simulink model "BEV_Components_OctNov24"  (R2024b)
settings: Solver=ode23tb  StartTime=0.0  StopTime=50  RelTol=1e-3
InitFcn:
  | P=150;
  | i_g=20;
  | Batt_C=90;
  | 
  | m=1200;
  | c=.28;
  | frr=0.014;
  | g=9.81;
  | Cmax=Batt_C*1e3/340;
  | et=0.9;
  | rw=.37;
libraries: simulink x1
settings Model: Creator=Kamyar  LastModifiedBy=samar
settings SolverCC: AlgebraicLoopSolver=TrustRegion
settings DebuggingCC: UnconnectedInputMsg=warning  UnconnectedOutputMsg=warning  UnconnectedLineMsg=warning
settings ModelReferenceCC: EnableRefExpFcnMdlSchedulingChecks=on
settings RTWCC: GPUComputeCapability=3.5  DLArmComputeVersion=19.05

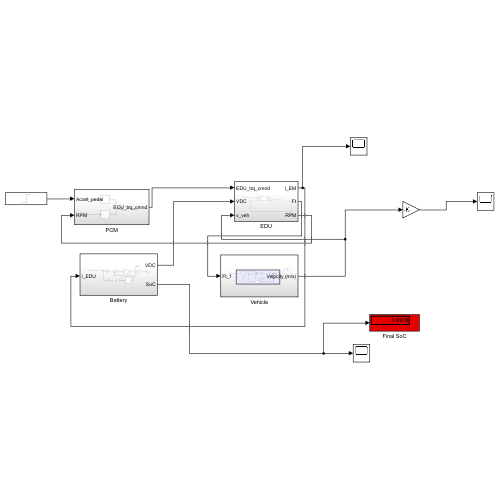
[thumbnail: Simulink's stored preview of the top-level diagram]
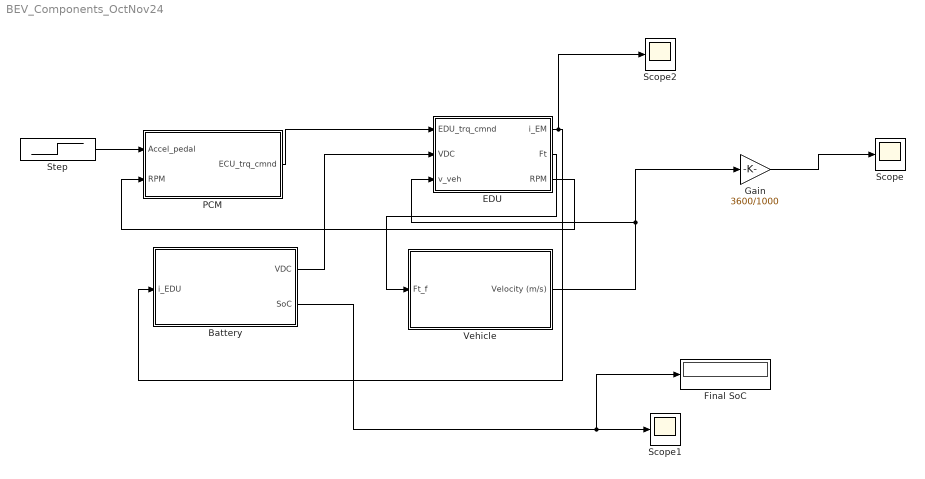
== system BEV_Components_OctNov24 ==
  Battery : Subsystem
  EDU : Subsystem
  Final SoC : Display
  Gain : Gain  Gain=3600/1000
  PCM : Subsystem
  Scope : Scope
  Scope1 : Scope
  Scope2 : Scope
  Step : Step  After=.6  SampleTime=0
  Vehicle : Subsystem
  wires:
  PCM/1(ECU_trq_cmnd) -> EDU/1(EDU_trq_cmnd)
  EDU/3(RPM) -> PCM/2(RPM)
  EDU/1(i_EM) -> Scope2/1, Battery/1(i_EDU)
  EDU/2(Ft) -> Vehicle/1(Ft_f)
  Battery/1(VDC) -> EDU/2(VDC)
  Vehicle/1(Velocity (m/s)) -> Gain/1, EDU/3(v_veh)
  Step/1 -> PCM/1(Accel_pedal)
  Battery/2(SoC) -> Final SoC/1, Scope1/1
  Gain/1 -> Scope/1

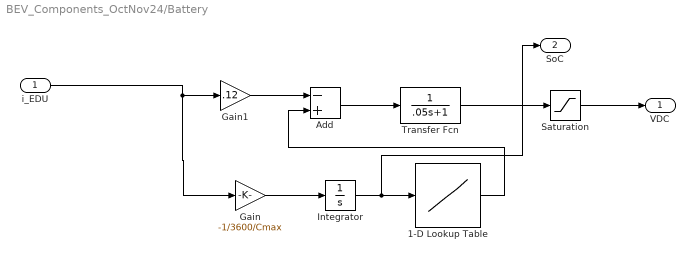
== system BEV_Components_OctNov24/Battery ==
  i_EDU : Inport
  1-D Lookup Table : Lookup_n-D  NumberOfTableDimensions=1  BreakpointsForDimension1=|  Table=|  InternalRulePriority=Speed  RndMeth=Simplest
      BreakpointsForDimension1=|
      | [0
      | 0.028708134
      | 0.04784689
      | 0.105263158
      | 0.207336523
      | 0.398724083
      | 0.535885167
      | 0.596491228
      | 0.68261563
      | 0.797448166
      | 1
      | ]
      Table=|
      | [279.7468354
      | 298.9873418
      | 313.164557
      | 323.0379747
      | 330.6329114
      | 339.7468354
      | 344.556962
      | 347.8481013
      | 356.4556962
      | 367.0886076
      | 391.1392405
      | ]
  Add : Sum  Inputs=-+
  Gain : Gain  Gain=-1/3600/Cmax
  Gain1 : Gain  Gain=.12
  Integrator : Integrator  InitialCondition=1
  Saturation : Saturate  UpperLimit=inf  LowerLimit=200
  Transfer Fcn : TransferFcn  Denominator=[.05 1]
  VDC : Outport
  SoC : Outport  Port=2
  wires:
  i_EDU/1 -> Gain/1, Gain1/1
  Gain/1 -> Integrator/1
  Integrator/1 -> SoC/1, 1-D Lookup Table/1
  1-D Lookup Table/1 -> Add/2
  Gain1/1 -> Add/1
  Add/1 -> Transfer Fcn/1
  Transfer Fcn/1 -> Saturation/1
  Saturation/1 -> VDC/1

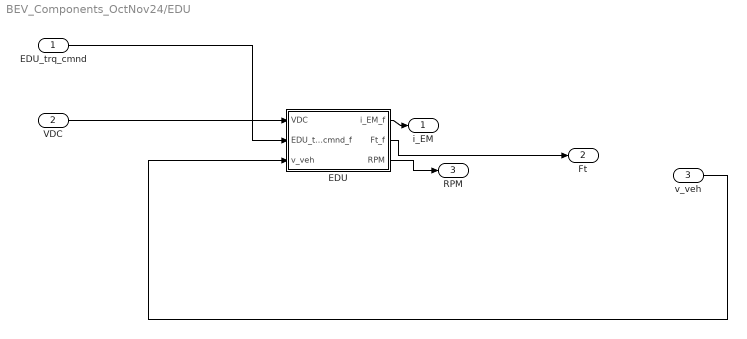
== system BEV_Components_OctNov24/EDU ==
  EDU_trq_cmnd : Inport
  VDC : Inport  Port=2
  v_veh : Inport  Port=3
  " EDU" : Subsystem
  i_EM : Outport
  Ft : Outport  Port=2
  RPM : Outport  Port=3
  wires:
  " EDU"/2(Ft_f) -> Ft/1
  VDC/1 -> " EDU"/1(VDC)
  v_veh/1 -> " EDU"/3(v_veh)
  " EDU"/1(i_EM_f) -> i_EM/1
  EDU_trq_cmnd/1 -> " EDU"/2(EDU_trq_cmnd_f)
  " EDU"/3(RPM) -> RPM/1

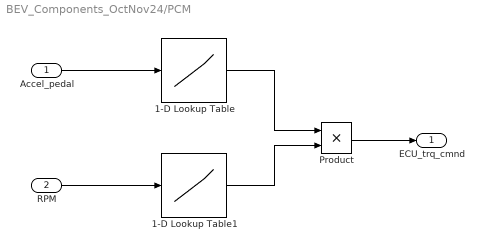
== system BEV_Components_OctNov24/PCM ==
  Accel_pedal : Inport
  RPM : Inport  Port=2
  1-D Lookup Table : Lookup_n-D  NumberOfTableDimensions=1  BreakpointsForDimension1=0:.2:1  Table=[0 .4 .6 .825 .95 1]  InternalRulePriority=Speed  RndMeth=Simplest
  1-D Lookup Table1 : Lookup_n-D  NumberOfTableDimensions=1  BreakpointsForDimension1=[0:500:13000]  Table=[ones(1,9)*P*1e3/4000/(pi/30),P*1e3/(pi/30)./[4500:500:13000]]  InternalRulePriority=Speed  RndMeth=Simplest
  Product : Product
  ECU_trq_cmnd : Outport
  wires:
  Accel_pedal/1 -> 1-D Lookup Table/1
  1-D Lookup Table1/1 -> Product/2
  1-D Lookup Table/1 -> Product/1
  Product/1 -> ECU_trq_cmnd/1
  RPM/1 -> 1-D Lookup Table1/1

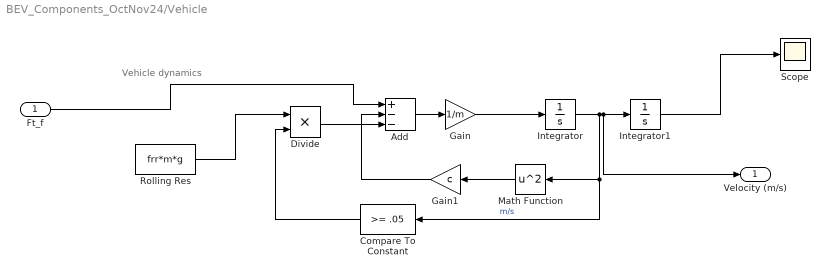
== system BEV_Components_OctNov24/Vehicle ==
  note: Vehicle dynamics
  Ft_f : Inport
  Add : Sum  Inputs=+--
  Compare To Constant : simulink/Logic and Bit Operations/Compare To Constant  relop=>=  const=.05  OutDataTypeStr=boolean
  Divide : Product
  Gain : Gain  Gain=1/m
  Gain1 : Gain  Gain=c
  Integrator : Integrator
  Integrator1 : Integrator
  Math Function : Math  Operator=square
  Rolling Res : Constant  Value=frr*m*g
  Scope : Scope
  Velocity (m/s) : Outport
  wires:
  Compare To Constant/1 -> Divide/2
  Rolling Res/1 -> Divide/1
  Divide/1 -> Add/3
  Gain/1 -> Integrator/1
  Add/1 -> Gain/1
  Gain1/1 -> Add/2
  Integrator/1 -> Compare To Constant/1, Math Function/1, Velocity (m/s)/1, Integrator1/1  "m/s"
  Math Function/1 -> Gain1/1
  Ft_f/1 -> Add/1
  Integrator1/1 -> Scope/1

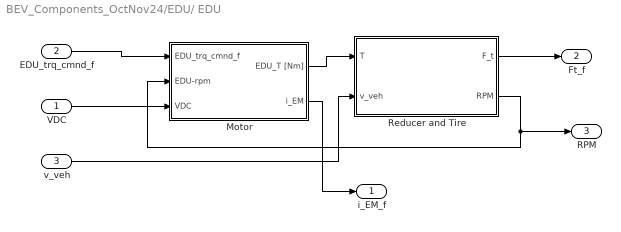
== system BEV_Components_OctNov24/EDU/ EDU ==
  VDC : Inport
  EDU_trq_cmnd_f : Inport  Port=2
  v_veh : Inport  Port=3
  Motor : Subsystem
  Reducer and Tire : Subsystem
  i_EM_f : Outport
  Ft_f : Outport  Port=2
  RPM : Outport  Port=3
  wires:
  Motor/2(i_EM) -> i_EM_f/1
  Reducer and Tire/1(F_t) -> Ft_f/1
  Reducer and Tire/2(RPM) -> RPM/1, Motor/2(EDU-rpm)
  v_veh/1 -> Reducer and Tire/2(v_veh)
  Motor/1(EDU_T [Nm]) -> Reducer and Tire/1(T)
  VDC/1 -> Motor/3(VDC)
  EDU_trq_cmnd_f/1 -> Motor/1(EDU_trq_cmnd_f)

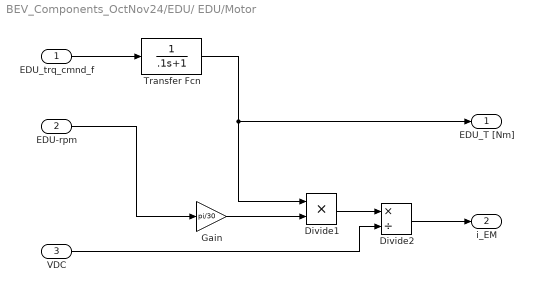
== system BEV_Components_OctNov24/EDU/ EDU/Motor ==
  EDU_trq_cmnd_f : Inport
  EDU-rpm : Inport  Port=2
  VDC : Inport  Port=3
  Divide1 : Product
  Divide2 : Product  Inputs=*/
  Gain : Gain  Gain=pi/30
  Transfer Fcn : TransferFcn  Denominator=[.1 1]
  EDU_T [Nm] : Outport
  i_EM : Outport  Port=2
  wires:
  EDU-rpm/1 -> Gain/1
  EDU_trq_cmnd_f/1 -> Transfer Fcn/1
  Divide1/1 -> Divide2/1
  Divide2/1 -> i_EM/1
  VDC/1 -> Divide2/2
  Gain/1 -> Divide1/2
  Transfer Fcn/1 -> Divide1/1, EDU_T [Nm]/1

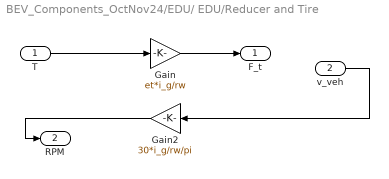
== system BEV_Components_OctNov24/EDU/ EDU/Reducer and Tire ==
  T : Inport
  v_veh : Inport  Port=2
  Gain : Gain  Gain=et*i_g/rw
  Gain2 : Gain  Gain=30*i_g/rw/pi
  F_t : Outport
  RPM : Outport  Port=2
  wires:
  Gain2/1 -> RPM/1
  T/1 -> Gain/1
  v_veh/1 -> Gain2/1
  Gain/1 -> F_t/1
